simulink model "temp_chamber"  (R2025a)
settings: Solver=VariableStepAuto  StartTime=0.0  StopTime=4000.0  RelTol=1e-3
settings Model: Creator=Laurenpearse  LastModifiedBy=Laurenpearse

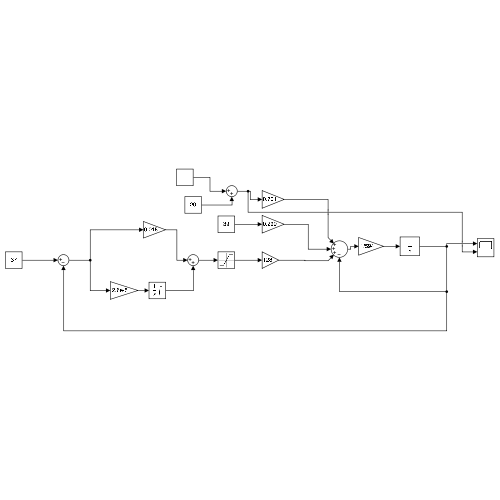
[thumbnail: Simulink's stored preview of the top-level diagram]
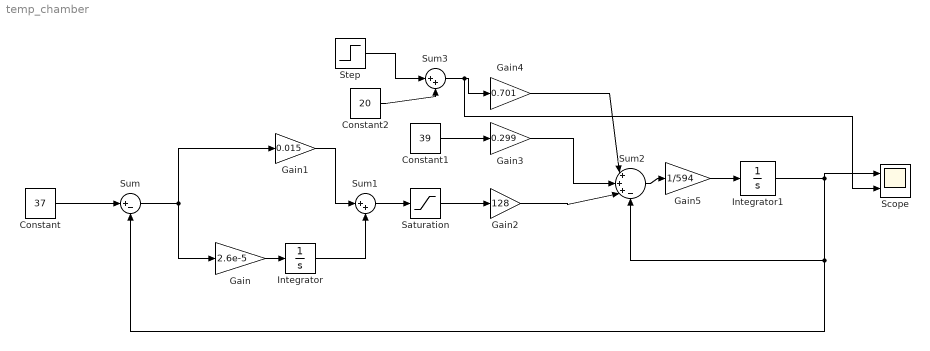
== system temp_chamber ==
  Constant : Constant  Value=37
  Constant1 : Constant  Value=39
  Constant2 : Constant  Value=20
  Gain : Gain  Gain=2.6e-5
  Gain1 : Gain  Gain=0.015
  Gain2 : Gain  Gain=128
  Gain3 : Gain  Gain=0.299
  Gain4 : Gain  Gain=0.701
  Gain5 : Gain  Gain=1/594
  Integrator : Integrator  LimitOutput=on  UpperSaturationLimit=1  LowerSaturationLimit=0
  Integrator1 : Integrator  InitialCondition=22
  Saturation : Saturate  UpperLimit=1  LowerLimit=0
  Scope : Scope  NumInputPorts=2
      settings: ActiveDisplayYMinimum=9.816346668586597  ActiveDisplayYMaximum=46.93494470756383
  Step : Step  Time=2500  After=-4  SampleTime=0
  Sum : Sum  Inputs=|+-
  Sum1 : Sum  Inputs=|++
  Sum2 : Sum  Inputs=|+++-
  Sum3 : Sum  Inputs=|++
  wires:
  Sum1/1 -> Saturation/1
  Gain/1 -> Integrator/1
  Constant/1 -> Sum/1
  Saturation/1 -> Gain2/1
  Constant1/1 -> Gain3/1
  Gain4/1 -> Sum2/1
  Gain3/1 -> Sum2/2
  Gain2/1 -> Sum2/3
  Sum2/1 -> Gain5/1
  Gain5/1 -> Integrator1/1
  Integrator1/1 -> Sum2/4, Sum/2, Scope/1
  Integrator/1 -> Sum1/2
  Gain1/1 -> Sum1/1
  Sum/1 -> Gain1/1, Gain/1
  Constant2/1 -> Sum3/2
  Step/1 -> Sum3/1
  Sum3/1 -> Scope/2, Gain4/1
